simulink model "IntegratedSatelliteControl"  (R2026a)
settings: Solver=FixedStepDiscrete  StopTime=c.T  FixedStep=c.dt
InitFcn:
  | if ~exist('c','var'), c=isc_tracking_config; end
model workspace (MAT data in the model file):
  c.mode = 'optical_event'
  c.scenario = 'pointing'
  c.seed = 11
  c.dt = 0.05
  c.T = 75
  c.N = 4
  c.faultStart = 25
  c.faultEnd = 60
  c.positions = [0  1000  1000  0; 0  0  1000  1000; 0  0  0  0]
  c.edges = [1  2; 1  3; 1  4; 2  3; 2  4; 3  4]
  c.M = 12
  c.sender = [1 2 1 3 1 4 2 3 2 4 3 4]
  c.receiver = [2 1 3 1 4 1 3 2 4 2 4 3]
  c.J = [0.03  0  0; 0  0.025  0; 0  0  0.02]
  c.umax = 0.002
  c.kp = 0.0015
  c.kd = 0.01
  c.coupling = 0.65
  c.smc = 2e-06
  c.surfaceGain = 0.18
  c.boundary = 0.0003
  c.observerGain = 2
  c.divergence = 0.0003
  c.P0 = 1e-06
  c.sensitivity = 2e-07
  c.plantDivergenceScale = 1
  c.pointingFaultScale = 1
  c.gimbalTau = 0.06
  c.gimbalLimit = 0.1
  c.gimbalRate = 0.035
  c.powerNoise = 0.008
  c.probeAmplitude = 4.8e-05
  c.probeDwell = 0.4
  c.fitWindow = 2
  c.fitSamples = 40
  c.decisionSteps = 4
  c.maxCorrection = 0.00045
  c.delay = 0.1
  c.jitter = 0.1
  c.randomDrop = 0.02
  c.period = 0.2
  c.eventMin = 0.1
  c.eventMax = 0.8
  c.eventAngle = 0.00015
  c.eventRate = 0.0001
  c.staleLimit = 1.5
  c.ideal = 0
  c.recovery = 1
  c.event = 1
  c.predict = 1
  c.task = 'leader_tracking'
  c.parent = [0 1 2 3]
  c.activeEndpoints = [1 2 7 8 11 12]
  c.offsets = [1  0.999997000002  0.999997625001  0.999998250001; 0  0.001999998  -0.0014999988125  0.000999999416667; 0  -0.000999999  0.0014999988125  0.000499999708333; 0  0.000999999  0.000499999604167  -0.001499999125]
  c.policy = 'off'
  c.manageSchedule = 0
  c.managePrediction = 0
  c.managedHorizon = 3
  c.managedGap = 0.2
  c.infeasibleGap = 1.6
  c.blackout = 0
  c.referencePhase = 0
settings Model: Creator=rishi  LastModifiedBy=rishi

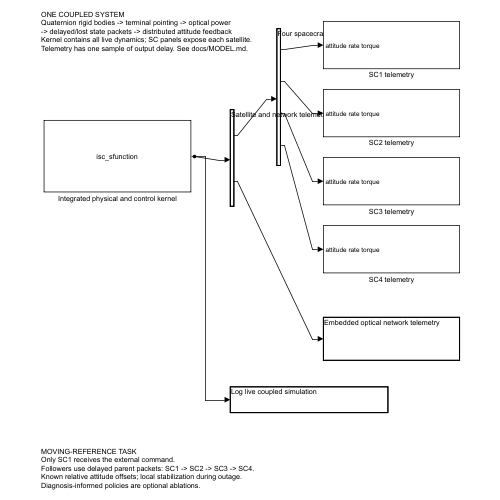
[thumbnail: Simulink's stored preview of the top-level diagram]
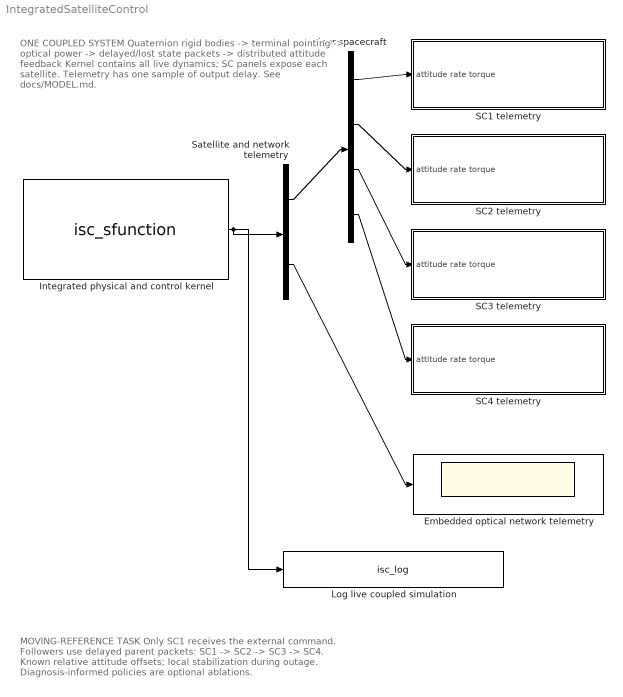
== system IntegratedSatelliteControl ==
  note: ONE COUPLED SYSTEM
      | Quaternion rigid bodies -> terminal pointing -> optical power
      | -> delayed/lost state packets -> distributed attitude feedback
      | Kernel contains all live dynamics; SC panels expose each satellite.
      | Telemetry has one sample of output delay. See docs/MODEL.md.
  note: MOVING-REFERENCE TASK
      | Only SC1 receives the external command.
      | Followers use delayed parent packets: SC1 -> SC2 -> SC3 -> SC4.
      | Known relative attitude offsets; local stabilization during outage.
      | Diagnosis-informed policies are optional ablations.
  Embedded optical network telemetry : Scope
  Four spacecraft : Demux  Outputs=[9 9 9 9]
  Integrated physical and control kernel : M-S-Function  FunctionName=isc_sfunction  Parameters=c
  Log live coupled simulation : ToWorkspace  VariableName=isc_log  SaveFormat=Timeseries  SampleTime=-1
  SC1 telemetry : Subsystem
  SC2 telemetry : Subsystem
  SC3 telemetry : Subsystem
  SC4 telemetry : Subsystem
  Satellite and network telemetry : Demux  Outputs=[36 84]
  wires:
  Integrated physical and control kernel/1 -> Satellite and network telemetry/1, Log live coupled simulation/1
  Satellite and network telemetry/1 -> Four spacecraft/1
  Four spacecraft/1 -> SC1 telemetry/1(attitude rate torque)
  Four spacecraft/2 -> SC2 telemetry/1(attitude rate torque)
  Four spacecraft/3 -> SC3 telemetry/1(attitude rate torque)
  Four spacecraft/4 -> SC4 telemetry/1(attitude rate torque)
  Satellite and network telemetry/2 -> Embedded optical network telemetry/1

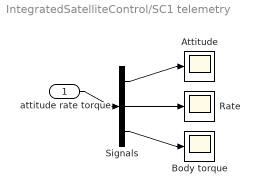
== system IntegratedSatelliteControl/SC1 telemetry ==
  attitude rate torque : Inport
  Attitude : Scope
  Body torque : Scope
  Rate : Scope
  Signals : Demux  Outputs=[3 3 3]
  wires:
  attitude rate torque/1 -> Signals/1
  Signals/1 -> Attitude/1
  Signals/2 -> Rate/1
  Signals/3 -> Body torque/1

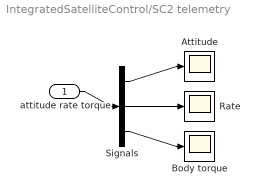
== system IntegratedSatelliteControl/SC2 telemetry ==
  attitude rate torque : Inport
  Attitude : Scope
  Body torque : Scope
  Rate : Scope
  Signals : Demux  Outputs=[3 3 3]
  wires:
  attitude rate torque/1 -> Signals/1
  Signals/1 -> Attitude/1
  Signals/2 -> Rate/1
  Signals/3 -> Body torque/1

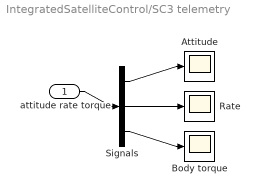
== system IntegratedSatelliteControl/SC3 telemetry ==
  attitude rate torque : Inport
  Attitude : Scope
  Body torque : Scope
  Rate : Scope
  Signals : Demux  Outputs=[3 3 3]
  wires:
  attitude rate torque/1 -> Signals/1
  Signals/1 -> Attitude/1
  Signals/2 -> Rate/1
  Signals/3 -> Body torque/1

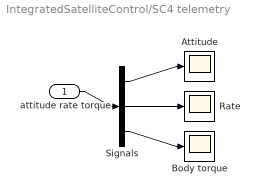
== system IntegratedSatelliteControl/SC4 telemetry ==
  attitude rate torque : Inport
  Attitude : Scope
  Body torque : Scope
  Rate : Scope
  Signals : Demux  Outputs=[3 3 3]
  wires:
  attitude rate torque/1 -> Signals/1
  Signals/1 -> Attitude/1
  Signals/2 -> Rate/1
  Signals/3 -> Body torque/1
